simulink model "finalmodel2"  (R2024b)
settings: Solver=ode4  StartTime=0.0  StopTime=110.0  FixedStep=SampleTime  MaxStep=1e-3  RelTol=1e-4  AbsTol=1e-3
values from neighbouring files (symbols this model uses):
  Cf = 0.00911825194797    [finalmodel2.mat]    (also in finalmodel3.mat)
  D = 6191.85011148    [finalmodel2.mat]    (also in finalmodel3.mat)
  J = 773.981263935    [finalmodel2.mat]    (also in finalmodel3.mat)
  k10 = 1    [finalmodel2.mat]    (also in finalmodel3.mat)
  k11 = 25    [finalmodel2.mat]    (also in finalmodel3.mat)
  k12 = 1    [finalmodel2.mat]    (also in finalmodel3.mat)
  k13 = 120    [finalmodel2.mat]    (also in finalmodel3.mat)
  k14 = 1    [finalmodel2.mat]    (also in finalmodel3.mat)
  k2 = 9.4    [finalmodel2.mat]    (also in finalmodel3.mat)
  k3 = 1    [finalmodel2.mat]    (also in finalmodel3.mat)
  k4 = 25    [finalmodel2.mat]    (also in finalmodel3.mat)
  k5 = 1    [finalmodel2.mat]    (also in finalmodel3.mat)
  k6 = 120    [finalmodel2.mat]    (also in finalmodel3.mat)
  k7 = 1    [finalmodel2.mat]    (also in finalmodel3.mat)
  k9 = 9.4    [finalmodel2.mat]    (also in finalmodel3.mat)
  Kip_vsg = 0.00606060606061    [finalmodel2.mat]    (also in finalmodel3.mat)
  Kq_vsg = 1.48453923805e-06    [finalmodel2.mat]    (also in finalmodel3.mat)
  Kvi_vsg = 899.93539556    [finalmodel2.mat]    (also in finalmodel3.mat)
  Kvp_vsg = 5.72916666667    [finalmodel2.mat]    (also in finalmodel3.mat)
  L1 = 1.15749049521e-05    [finalmodel2.mat]    (also in finalmodel3.mat)
  Ls = 1.92915082536e-06    [finalmodel2.mat]    (also in finalmodel3.mat)
  Pset = 8281000    [finalmodel2.mat]    (also in finalmodel3.mat = 8280000)
  R1 = 0.000290909090909    [finalmodel2.mat]    (also in finalmodel3.mat)
  SampleTime = 5e-05    [finalmodel2.mat]    (also in finalmodel3.mat)
  Us = 326.598632371    [finalmodel2.mat]    (also in finalmodel3.mat)
  Vdclink = 800    [finalmodel2.mat]    (also in finalmodel3.mat)
  wn = 376.991118431    [finalmodel2.mat]    (also in finalmodel3.mat)
undefined symbols (not defined in the file or in its folder): sigbuilder_block
libraries: spsThreePhaseVIMeasurementLib x15, spsLoadFlowBusLib x9, spsThreePhasePISectionLineLib x6, spsThreePhaseTransformerTwoWindingsLib x4, spsThreePhaseParallelRLCLoadLib x4, spsabctodq0Lib x4, spsThreePhaseSeriesRLCBranchLib x3, spsSynchronousMachinepuStandardLib x2, spsExcitationSystemLib x2, spsMultiBandPowerSystemStabilizerLib x2, spsSteamTurbineandGovernorLib x2, spsGroundLib x2
(part 3 of 3)

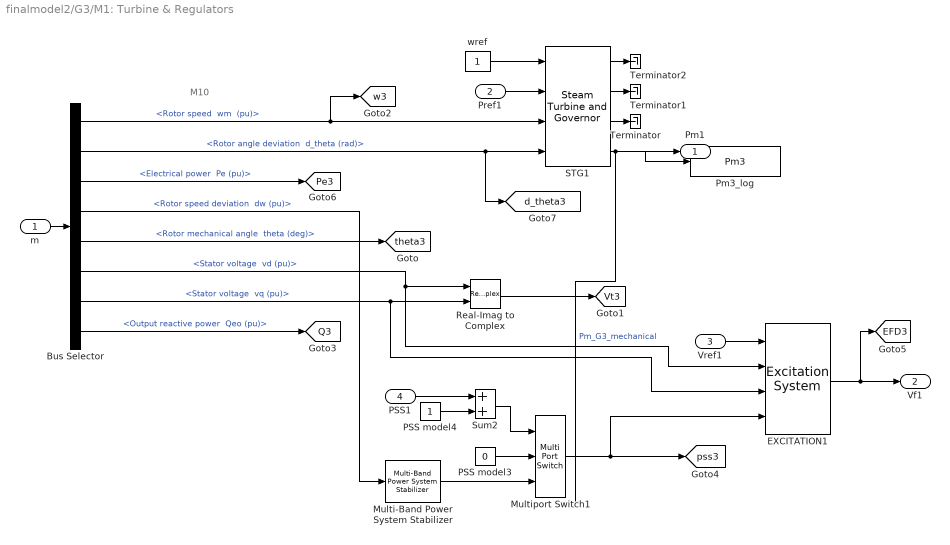
== system finalmodel2/G3/M1: Turbine & Regulators ==
  note: M10
  m : Inport  SampleTime=SampleTime
  Pref1 : Inport  Port=2  SampleTime=SampleTime
  Vref1 : Inport  Port=3  SampleTime=SampleTime
  PSS1 : Inport  Port=4  SampleTime=SampleTime
  Bus Selector : BusSelector  OutputSignals="Mechanical.Rotor speed  wm  (pu),Mechanical.Rotor angle deviation  d_theta (rad),Mechanical.Electrical power  Pe (pu),Mechanical.Rotor speed deviation  dw (pu),Mechanical.Rotor mechanical angle  theta (deg),dq0 components.Stator voltage  vd (pu),dq0 components.Stator voltage  vq (pu),Output reactive power  Qeo (pu)"
  EXCITATION1 : spsExcitationSystemLib/Excitation System  tr=0.01  reg=[20 .2]  exc=[ 1, 0.314 ]  tgr=[ 10 1]  damp=[ 0.063, 0.35 ]  sat=[ 0, 0 ]  lim="[ -5 5  0 ]"  v0=[1.025 1.2647]
      link override Model: Ts=SampleTime
      link override Model/Damping kfd.s // (tfd.s +1)/1st-Order Discrete Filter: Ts=SampleTime
      link override Model/Damping kfd.s // (tfd.s +1)/1st-Order Discrete Filter/Discrete State-Space: SampleTime=SampleTime
      link override Model/Exciter  1 // (te.s + ke)/1st order Lowpass: Ts=SampleTime
      link override Model/Exciter  1 // (te.s + ke)/1st order Lowpass/Discrete State-Space: SampleTime=SampleTime
      link override Model/Lead Lag Compensator tc.s+1 // tb.s+1: Ts=SampleTime
      link override Model/Lead Lag Compensator tc.s+1 // tb.s+1/Discrete State-Space: SampleTime=SampleTime
      link override Model/Low Pass Filter 1 // (tr.s +1) (with IC): Ts=SampleTime
      link override Model/Low Pass Filter 1 // (tr.s +1) (with IC)/Discrete State-Space: SampleTime=SampleTime
      link override Model/Main Regulator ka // (ta.s +1)/1st order Lowpass: Ts=SampleTime
      link override Model/Main Regulator ka // (ta.s +1)/1st order Lowpass/Discrete State-Space: SampleTime=SampleTime
      link override Model/Positive Sequence Voltage: Expr=sqrt(abs(u(1)^2 + u(2)^2))
      link override Model/Unit Delay1: SampleTime=SampleTime
      link override Model/Unit Delay2: SampleTime=SampleTime
      settings: LibrarySourceBlock=sps_lib/Electrical Machines/Synchronous Machine Control/Excitation System
  Multi-Band Power System Stabilizer : spsMultiBandPowerSystemStabilizerLib/Multi-Band Power System Stabilizer  OperationMode=Simplified settings  Kg=k1  GL=[k2 k3]  GI=[k4 k5]  GH=[k6 k7]  GLd=[66 66 9.4]  TcLF=[1.667 2 0 0 0 0 2 2.4 0 0 0 0 1 1]  GId=[66 66 47.6]  TcIF=[1 1 0.25 0.3 0 0 1 1 0.3 0.36 0 0 0 0]  GHd=[66 66 233]  TcHF="[0.01 0.012 0 0 0 0  0.012 0.0144 0 0 0 0 1 1]"  LIM=[.075 .15 .15 .15]  Plot_On=off  MagdB_On=off  FreqRange=logspace(-2,2,500)
      link override Model/Discrete Lead-Lag1: Ts=SampleTime
      link override Model/Discrete Lead-Lag1/Discrete State-Space: SampleTime=SampleTime
      link override Model/Discrete Lead-Lag2: Ts=SampleTime
      link override Model/Discrete Lead-Lag2/Discrete State-Space: SampleTime=SampleTime
      link override Model/Discrete Lead-Lag3: Ts=SampleTime
      link override Model/Discrete Lead-Lag3/Discrete State-Space: SampleTime=SampleTime
      link override Model/Discrete Lead-Lag4: Ts=SampleTime
      link override Model/Discrete Lead-Lag4/Discrete State-Space: SampleTime=SampleTime
      link override Model/Discrete Lead-Lag5: Ts=SampleTime
      link override Model/Discrete Lead-Lag5/Discrete State-Space: SampleTime=SampleTime
      link override Model/Discrete Lead-Lag6: Ts=SampleTime
      link override Model/Discrete Lead-Lag6/Discrete State-Space: SampleTime=SampleTime
      link override Model/HF speed sensor: Ts=SampleTime
      link override Model/HF speed sensor/Discrete State-Space: SampleTime=SampleTime
      link override Model/LF and IF speed sensor: Ts=SampleTime
      link override Model/LF and IF speed sensor/Discrete State-Space: SampleTime=SampleTime
      link override Model/Transfer function for detailed model (HF)/Transfer functions for detailed stabilizer/Discrete Lead-Lag1: Ts=SampleTime
      link override Model/Transfer function for detailed model (HF)/Transfer functions for detailed stabilizer/Discrete Lead-Lag1/Discrete State-Space: SampleTime=SampleTime
      link override Model/Transfer function for detailed model (HF)/Transfer functions for detailed stabilizer/Discrete Lead-Lag2: Ts=SampleTime
      link override Model/Transfer function for detailed model (HF)/Transfer functions for detailed stabilizer/Discrete Lead-Lag2/Discrete State-Space: SampleTime=SampleTime
      link override Model/Transfer function for detailed model (HF)/Transfer functions for detailed stabilizer1/Discrete Lead-Lag1: Ts=SampleTime
      link override Model/Transfer function for detailed model (HF)/Transfer functions for detailed stabilizer1/Discrete Lead-Lag1/Discrete State-Space: SampleTime=SampleTime
      link override Model/Transfer function for detailed model (HF)/Transfer functions for detailed stabilizer1/Discrete Lead-Lag2: Ts=SampleTime
      link override Model/Transfer function for detailed model (HF)/Transfer functions for detailed stabilizer1/Discrete Lead-Lag2/Discrete State-Space: SampleTime=SampleTime
      link override Model/Transfer function for detailed model (IF)/Transfer functions for detailed stabilizer/Discrete Lead-Lag1: Ts=SampleTime
      link override Model/Transfer function for detailed model (IF)/Transfer functions for detailed stabilizer/Discrete Lead-Lag1/Discrete State-Space: SampleTime=SampleTime
      link override Model/Transfer function for detailed model (IF)/Transfer functions for detailed stabilizer/Discrete Lead-Lag2: Ts=SampleTime
      link override Model/Transfer function for detailed model (IF)/Transfer functions for detailed stabilizer/Discrete Lead-Lag2/Discrete State-Space: SampleTime=SampleTime
      link override Model/Transfer function for detailed model (IF)/Transfer functions for detailed stabilizer1/Discrete Lead-Lag1: Ts=SampleTime
      link override Model/Transfer function for detailed model (IF)/Transfer functions for detailed stabilizer1/Discrete Lead-Lag1/Discrete State-Space: SampleTime=SampleTime
      link override Model/Transfer function for detailed model (IF)/Transfer functions for detailed stabilizer1/Discrete Lead-Lag2: Ts=SampleTime
      link override Model/Transfer function for detailed model (IF)/Transfer functions for detailed stabilizer1/Discrete Lead-Lag2/Discrete State-Space: SampleTime=SampleTime
      link override Model/Transfer function for detailed model (LF)/Transfer functions for detailed stabilizer/Discrete Lead-Lag1: Ts=SampleTime
      link override Model/Transfer function for detailed model (LF)/Transfer functions for detailed stabilizer/Discrete Lead-Lag1/Discrete State-Space: SampleTime=SampleTime
      link override Model/Transfer function for detailed model (LF)/Transfer functions for detailed stabilizer/Discrete Lead-Lag2: Ts=SampleTime
      link override Model/Transfer function for detailed model (LF)/Transfer functions for detailed stabilizer/Discrete Lead-Lag2/Discrete State-Space: SampleTime=SampleTime
      link override Model/Transfer function for detailed model (LF)/Transfer functions for detailed stabilizer1/Discrete Lead-Lag1: Ts=SampleTime
      link override Model/Transfer function for detailed model (LF)/Transfer functions for detailed stabilizer1/Discrete Lead-Lag1/Discrete State-Space: SampleTime=SampleTime
      link override Model/Transfer function for detailed model (LF)/Transfer functions for detailed stabilizer1/Discrete Lead-Lag2: Ts=SampleTime
      link override Model/Transfer function for detailed model (LF)/Transfer functions for detailed stabilizer1/Discrete Lead-Lag2/Discrete State-Space: SampleTime=SampleTime
      settings: LibrarySourceBlock=|
      | sps_lib/Electrical Machines/Synchronous Machine Control/Multi-Band
      | Power System Stabilizer
  Multiport Switch1 : MultiPortSwitch  Inputs=2  SampleTime=SampleTime  SaturateOnIntegerOverflow=off
  PSS model3 : Constant  Value=0  SampleTime=SampleTime
  PSS model4 : Constant  SampleTime=SampleTime
  Pm3_log : ToWorkspace  VariableName=Pm3  SaveFormat=Timeseries  SampleTime=-1
  Real-Imag to Complex : RealImagToComplex  SampleTime=SampleTime
  STG1 : spsSteamTurbineandGovernorLib/Steam Turbine and Governor  gentype=Tandem-compound (single mass)  reg1="[ 1  0.05    0 ]"  reg2="[ 0.001  0.15 ]"  reg3="[ -0.1  0.1  0  4.496 ]"  N=3600  turb1="[ 0  10   3.3   0.5   ]"  turb2="[   0   0.36    0.36   0.28   ]"  HA="[ 0.046  1.430  1.465   0.192 ]"  KA="[ 90.44  53.88  64.59   62.94  ]"  DA="[ 0.0115  0.3575  0.3663   0.0137  ]"  ini1=0.66512  ini2=[0.779316,-31.4247]
      link override Model/4 mass shaft/1 mass/Mass2: Ts=SampleTime
      link override Model/4 mass shaft/1 mass/Mass2/Ad*x(k-1): SampleTime=SampleTime
      link override Model/4 mass shaft/1 mass/Mass2/Bd*(u(k)+ u(k-1)): SampleTime=SampleTime
      link override Model/4 mass shaft/1 mass/Mass2/Delay_u: SampleTime=SampleTime
      link override Model/4 mass shaft/1 mass/Mass2/Delay_x: SampleTime=SampleTime
      link override Model/4 mass shaft/1 mass/Mass2/Digital Clock: SampleTime=SampleTime
      link override Model/4 mass shaft/1 mass/Mass2/Prediction/Unit Delay3: SampleTime=SampleTime
      link override Model/4 mass shaft/2 masses/Mass2: Ts=SampleTime
      link override Model/4 mass shaft/2 masses/Mass2/Ad*x(k-1): SampleTime=SampleTime
      link override Model/4 mass shaft/2 masses/Mass2/Bd*(u(k)+ u(k-1)): SampleTime=SampleTime
      link override Model/4 mass shaft/2 masses/Mass2/Delay_u: SampleTime=SampleTime
      link override Model/4 mass shaft/2 masses/Mass2/Delay_x: SampleTime=SampleTime
      link override Model/4 mass shaft/2 masses/Mass2/Digital Clock: SampleTime=SampleTime
      link override Model/4 mass shaft/2 masses/Mass2/Prediction/Unit Delay3: SampleTime=SampleTime
      link override Model/4 mass shaft/2 masses/Mass3: Ts=SampleTime
      link override Model/4 mass shaft/2 masses/Mass3/Ad*x(k-1): SampleTime=SampleTime
      link override Model/4 mass shaft/2 masses/Mass3/Bd*(u(k)+ u(k-1)): SampleTime=SampleTime
      link override Model/4 mass shaft/2 masses/Mass3/Delay_u: SampleTime=SampleTime
      link override Model/4 mass shaft/2 masses/Mass3/Delay_x: SampleTime=SampleTime
      link override Model/4 mass shaft/2 masses/Mass3/Digital Clock: SampleTime=SampleTime
      link override Model/4 mass shaft/2 masses/Mass3/Prediction/Unit Delay3: SampleTime=SampleTime
      link override Model/4 mass shaft/3 masses/Mass2: Ts=SampleTime
      link override Model/4 mass shaft/3 masses/Mass2/Ad*x(k-1): SampleTime=SampleTime
      link override Model/4 mass shaft/3 masses/Mass2/Bd*(u(k)+ u(k-1)): SampleTime=SampleTime
      link override Model/4 mass shaft/3 masses/Mass2/Delay_u: SampleTime=SampleTime
      link override Model/4 mass shaft/3 masses/Mass2/Delay_x: SampleTime=SampleTime
      link override Model/4 mass shaft/3 masses/Mass2/Digital Clock: SampleTime=SampleTime
      link override Model/4 mass shaft/3 masses/Mass2/Prediction/Unit Delay3: SampleTime=SampleTime
      link override Model/4 mass shaft/3 masses/Mass3: Ts=SampleTime
      link override Model/4 mass shaft/3 masses/Mass3/Ad*x(k-1): SampleTime=SampleTime
      link override Model/4 mass shaft/3 masses/Mass3/Bd*(u(k)+ u(k-1)): SampleTime=SampleTime
      link override Model/4 mass shaft/3 masses/Mass3/Delay_u: SampleTime=SampleTime
      link override Model/4 mass shaft/3 masses/Mass3/Delay_x: SampleTime=SampleTime
      link override Model/4 mass shaft/3 masses/Mass3/Digital Clock: SampleTime=SampleTime
      link override Model/4 mass shaft/3 masses/Mass3/Prediction/Unit Delay3: SampleTime=SampleTime
      link override Model/4 mass shaft/3 masses/Mass4: Ts=SampleTime
      link override Model/4 mass shaft/3 masses/Mass4/Ad*x(k-1): SampleTime=SampleTime
      link override Model/4 mass shaft/3 masses/Mass4/Bd*(u(k)+ u(k-1)): SampleTime=SampleTime
      link override Model/4 mass shaft/3 masses/Mass4/Delay_u: SampleTime=SampleTime
      link override Model/4 mass shaft/3 masses/Mass4/Delay_x: SampleTime=SampleTime
      link override Model/4 mass shaft/3 masses/Mass4/Digital Clock: SampleTime=SampleTime
      link override Model/4 mass shaft/3 masses/Mass4/Prediction/Unit Delay3: SampleTime=SampleTime
      link override Model/4 mass shaft/4 masses/Mass2: Ts=SampleTime
      link override Model/4 mass shaft/4 masses/Mass2/Ad*x(k-1): SampleTime=SampleTime
      link override Model/4 mass shaft/4 masses/Mass2/Bd*(u(k)+ u(k-1)): SampleTime=SampleTime
      link override Model/4 mass shaft/4 masses/Mass2/Delay_u: SampleTime=SampleTime
      link override Model/4 mass shaft/4 masses/Mass2/Delay_x: SampleTime=SampleTime
      link override Model/4 mass shaft/4 masses/Mass2/Digital Clock: SampleTime=SampleTime
      link override Model/4 mass shaft/4 masses/Mass2/Prediction/Unit Delay3: SampleTime=SampleTime
      link override Model/4 mass shaft/4 masses/Mass3: Ts=SampleTime
      link override Model/4 mass shaft/4 masses/Mass3/Ad*x(k-1): SampleTime=SampleTime
      link override Model/4 mass shaft/4 masses/Mass3/Bd*(u(k)+ u(k-1)): SampleTime=SampleTime
      link override Model/4 mass shaft/4 masses/Mass3/Delay_u: SampleTime=SampleTime
      link override Model/4 mass shaft/4 masses/Mass3/Delay_x: SampleTime=SampleTime
      link override Model/4 mass shaft/4 masses/Mass3/Digital Clock: SampleTime=SampleTime
      link override Model/4 mass shaft/4 masses/Mass3/Prediction/Unit Delay3: SampleTime=SampleTime
      link override Model/4 mass shaft/4 masses/Mass4: Ts=SampleTime
      link override Model/4 mass shaft/4 masses/Mass4/Ad*x(k-1): SampleTime=SampleTime
      link override Model/4 mass shaft/4 masses/Mass4/Bd*(u(k)+ u(k-1)): SampleTime=SampleTime
      link override Model/4 mass shaft/4 masses/Mass4/Delay_u: SampleTime=SampleTime
      link override Model/4 mass shaft/4 masses/Mass4/Delay_x: SampleTime=SampleTime
      link override Model/4 mass shaft/4 masses/Mass4/Digital Clock: SampleTime=SampleTime
      link override Model/4 mass shaft/4 masses/Mass4/Prediction/Unit Delay3: SampleTime=SampleTime
      link override Model/4 mass shaft/4 masses/Mass5: Ts=SampleTime
      link override Model/4 mass shaft/4 masses/Mass5/Ad*x(k-1): SampleTime=SampleTime
      link override Model/4 mass shaft/4 masses/Mass5/Bd*(u(k)+ u(k-1)): SampleTime=SampleTime
      link override Model/4 mass shaft/4 masses/Mass5/Delay_u: SampleTime=SampleTime
      link override Model/4 mass shaft/4 masses/Mass5/Delay_x: SampleTime=SampleTime
      link override Model/4 mass shaft/4 masses/Mass5/Digital Clock: SampleTime=SampleTime
      link override Model/4 mass shaft/4 masses/Mass5/Prediction/Unit Delay3: SampleTime=SampleTime
      link override Model/speed regulator/Servo-motor Position: SampleTime=SampleTime
      link override Model/speed regulator/Speed Relay: Ts=SampleTime
      link override Model/speed regulator/Speed Relay/In: SampleTime=SampleTime
      link override Model/speed regulator/Speed Relay/Model/Delay_x: SampleTime=SampleTime
      link override Model/speed regulator/Speed Relay/Out: SampleTime=SampleTime
      link override Model/steam turbine/Stage 1/Constant4: SampleTime=SampleTime
      link override Model/steam turbine/Stage 1/Stage1/Stage1: Ts=SampleTime
      link override Model/steam turbine/Stage 1/Stage1/Stage1/In: SampleTime=SampleTime
      link override Model/steam turbine/Stage 1/Stage1/Stage1/Model/Delay_x: SampleTime=SampleTime
      link override Model/steam turbine/Stage 1/Stage1/Stage1/Out: SampleTime=SampleTime
      link override Model/steam turbine/Stage 2 /Constant3: SampleTime=SampleTime
      link override Model/steam turbine/Stage 2 /Stage2/Stage2: Ts=SampleTime
      link override Model/steam turbine/Stage 2 /Stage2/Stage2/In: SampleTime=SampleTime
      link override Model/steam turbine/Stage 2 /Stage2/Stage2/Model/Delay_x: SampleTime=SampleTime
      link override Model/steam turbine/Stage 2 /Stage2/Stage2/Out: SampleTime=SampleTime
      link override Model/steam turbine/Stage 3/Constant2: SampleTime=SampleTime
      link override Model/steam turbine/Stage 3/Stage3/Stage3: Ts=SampleTime
      link override Model/steam turbine/Stage 3/Stage3/Stage3/In: SampleTime=SampleTime
      link override Model/steam turbine/Stage 3/Stage3/Stage3/Model/Delay_x: SampleTime=SampleTime
      link override Model/steam turbine/Stage 3/Stage3/Stage3/Out: SampleTime=SampleTime
      link override Model/steam turbine/Stage 4/Constant1: SampleTime=SampleTime
      link override Model/steam turbine/Stage 4/Stage4/Stage4: Ts=SampleTime
      link override Model/steam turbine/Stage 4/Stage4/Stage4/In: SampleTime=SampleTime
      link override Model/steam turbine/Stage 4/Stage4/Stage4/Model/Delay_x: SampleTime=SampleTime
      link override Model/steam turbine/Stage 4/Stage4/Stage4/Out: SampleTime=SampleTime
      settings: LibrarySourceBlock=|
      | sps_lib/Electrical Machines/Synchronous Machine Control/Steam Turbine
      | and Governor
  Sum2 : Sum  InputSameDT=on  SaturateOnIntegerOverflow=on  SampleTime=SampleTime  OutDataTypeStr=Inherit: Same as first input
  Terminator : Terminator
  Terminator1 : Terminator
  Terminator2 : Terminator
  wref : Constant  SampleTime=SampleTime
  Pm1 : Outport  SampleTime=SampleTime  InitialOutput=0
  Vf1 : Outport  Port=2  SampleTime=SampleTime  InitialOutput=0
  tag scope: EFD3=global, Pe3=global, Q3=global, Vt3=global, d_theta3=global, pss3=global, theta3=global, w3=global
  wires:
  Bus Selector/4 -> Multi-Band Power System Stabilizer/1  "<Rotor speed deviation  dw (pu)>"
  Multiport Switch1/1 -> EXCITATION1/4, [pss3]
  PSS model3/1 -> Multiport Switch1/2
  Multi-Band Power System Stabilizer/1 -> Multiport Switch1/3
  PSS model4/1 -> Sum2/2
  Sum2/1 -> Multiport Switch1/1
  PSS1/1 -> Sum2/1
  Bus Selector/8 -> [Q3]  "<Output reactive power  Qeo (pu)>"
  Bus Selector/3 -> [Pe3]  "<Electrical power  Pe (pu)>"
  Bus Selector/2 -> STG1/4, [d_theta3]  "<Rotor angle deviation  d_theta (rad)>"
  Bus Selector/1 -> STG1/3, [w3]  "<Rotor speed  wm  (pu)>"
  STG1/1 -> Terminator2/1
  STG1/2 -> Terminator1/1
  STG1/3 -> Terminator/1
  Bus Selector/6 -> EXCITATION1/2, Real-Imag to Complex/1  "<Stator voltage  vd (pu)>"
  Bus Selector/5 -> [theta3]  "<Rotor mechanical angle  theta (deg)>"
  Real-Imag to Complex/1 -> [Vt3]
  EXCITATION1/1 -> [EFD3], Vf1/1
  Vref1/1 -> EXCITATION1/1
  m/1 -> Bus Selector/1
  Pref1/1 -> STG1/2
  wref/1 -> STG1/1
  Bus Selector/7 -> Real-Imag to Complex/2, EXCITATION1/3  "<Stator voltage  vq (pu)>"
  STG1/4 -> Pm1/1, Pm3_log/1  "Pm_G3_mechanical"
